simulink model "wscc9_lfc_governor"  (R2024b)
settings: Solver=VariableStepAuto  StartTime=0.0  StopTime=60  MaxStep=0.01  RelTol=1e-3
InitFcn:
  | wscc9_lfc_init
values from neighbouring files (symbols this model uses):
  D = 4    [wscc9_lfc_init.m]
  D10 = del(1)    [wscc9_transient_init.m]
  D20 = del(2)    [wscc9_transient_init.m]
  D30 = del(3)    [wscc9_transient_init.m]
  E1 = E(1)    [wscc9_transient_init.m]
  E2 = E(2)    [wscc9_transient_init.m]
  E3 = E(3)    [wscc9_transient_init.m]
  f = 60    [wscc9_transient_init.m]
  H = [23.645 ; 6.4 ; 3.01]    [wscc9_transient_init.m]
  kS = S_MVA / S_base    [wscc9_lfc_init.m]
  Pm0 = Pe0    [wscc9_lfc_init.m]
  R = 0.05    [wscc9_lfc_init.m]    (also in wscc9_transient_init.m = linedataa(:,3))
  S_base = 100    [wscc9_lfc_init.m]
  t_step = 1    [wscc9_lfc_init.m]
  Tg = 0.2    [wscc9_lfc_init.m]
  Tt = 0.5    [wscc9_lfc_init.m]
  ws = 2*pi*f    [wscc9_lfc_init.m]
  Ypost = kron_reduce(Ystep, 3)    [wscc9_lfc_init.m]
  Ypre = Y1    [wscc9_lfc_init.m]
Description:
  | WSCC 3-machine 9-bus system: load-frequency study (classical SG, model 0.0, with a simple governor)
  | Run: wscc9_lfc_plot (simulates and plots), or press Run. InitFcn = wscc9_lfc_init.m sets every parameter.
  | Units: powers in pu on 100 MVA (MW in the measurement area), dw in rad/s, delta in rad, f in Hz.
  | Swing equation (each SG): d(dw)/dt = (pi f / H)(Pm - Pe - D kS dw/ws),   d(delta)/dt = dw
  | Governor (each SG): dPm = -(kS / R)(dw/ws) -> 1/(1 + s Tg) -> 1/(1 + s Tt),   Pm = Pm0 + dPm   (R = 0.05, Tg = 0.2 s, Tt = 0.5 s, D = 4)
  | Network: Pe_k = sum_j E_k E_j |Y_kj| cos(theta_kj - delta_k + delta_j);  Y switches from Ypre to Ypost at t_step (load step dP_L_MW at step_bus).
  | Goto/From tags: del1-3 = rotor angles, Pe1pre/Pe1post... = Pe before/after the step, w1-3 = dw, Pm1-3, Pe1-3 = measurement taps.
settings Model: Creator=Hussain  LastModifiedBy=Hussain
settings SolverCC: AlgebraicLoopSolver=TrustRegion
settings DebuggingCC: UnconnectedInputMsg=warning  UnconnectedOutputMsg=warning  UnconnectedLineMsg=warning  ArithmeticOperatorsInVariantConditions=warning
settings ModelReferenceCC: EnableRefExpFcnMdlSchedulingChecks=on
settings SFSimCC: SimUseLocalCustomCode=off  CustomCodeUndefinedFunction=UseInterfaceOnly
settings RTWCC: RTWUseLocalCustomCode=off  GPUComputeCapability=3.5
settings CodeAppCC: StateflowObjectComments=on

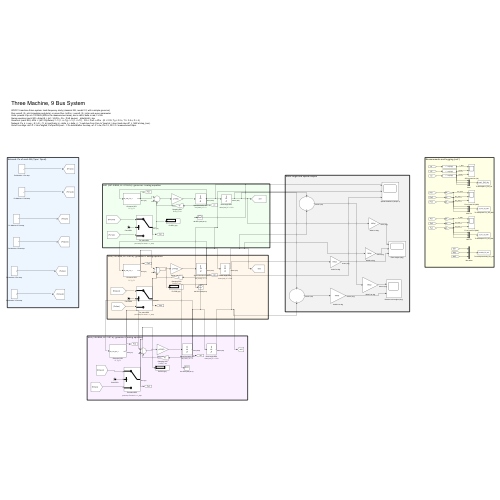
[thumbnail: Simulink's stored preview of the top-level diagram]
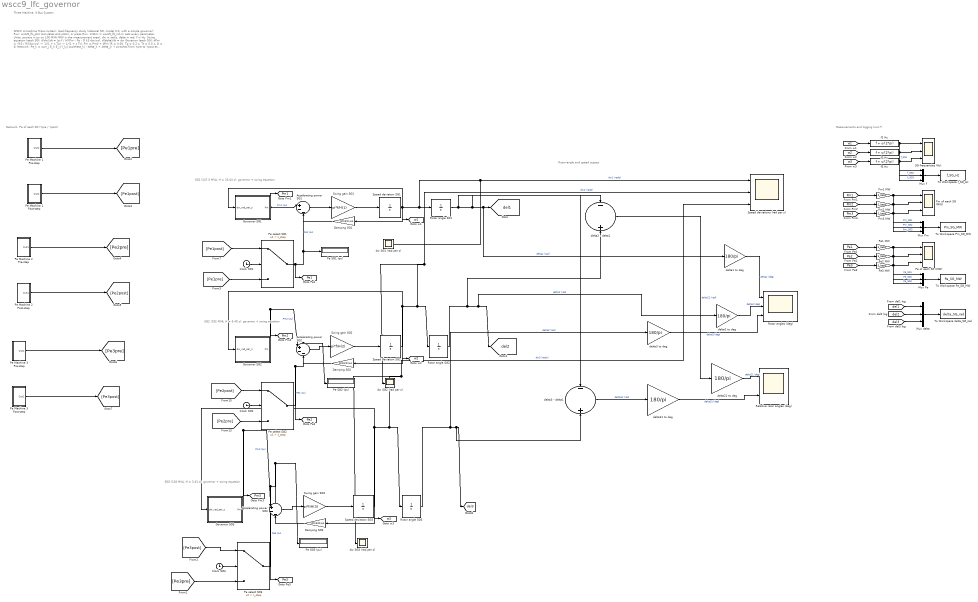
== system wscc9_lfc_governor ==
  note: Three Machine, 9 Bus System
  note: Network: Pe of each SG (Ypre / Ypost)
  note: SG1 (247.5 MVA, H = 23.64 s): governor + swing equation
  note: SG2 (192 MVA, H = 6.40 s): governor + swing equation
  note: SG3 (128 MVA, H = 3.01 s): governor + swing equation
  note: Rotor-angle and speed scopes
  note: Measurements and logging (out.*)
  note: WSCC 3-machine 9-bus system: load-frequency study (classical SG, model 0.0, with a simple governor)
      | Run: wscc9_lfc_plot (simulates and plots), or press Run. InitFcn = wscc9_lfc_init.m sets every parameter.
      | Units: powers in pu on 100 MVA (MW in the measurement area), dw in rad/s, delta in rad, f in Hz.
      | Swing equation (each SG): d(dw)/dt = (pi f / H)(Pm - Pe - D kS dw/ws),   d(delta)/dt = dw
      | Governor (each SG): dPm = -(kS / R)(dw/ws) -> 1/(1 + s Tg) -> 1/(1 + s Tt),   Pm = Pm0 + dPm   (R = 0.05, Tg = 0.2 s, Tt = 0.5 s, D = 4)
      | Network: Pe_k = sum_j E_k E_j |Y_kj| cos(theta_kj - delta_k + delta_j);  Y switches from Ypre to Ypost at t_step (load step dP_L_MW at step_bus).
      | Goto/From tags: del1-3 = rotor angles, Pe1pre/Pe1post... = Pe before/after the step, w1-3 = dw, Pm1-3, Pe1-3 = measurement taps.
  Accelerating power SG1 : Sum  Inputs=|+--
  Accelerating power SG2 : Sum  Inputs=|+--
  Accelerating power SG3 : Sum  Inputs=|+--
  Clock SG1 : Clock
  Clock SG2 : Clock
  Clock SG3 : Clock
  Damping SG1 : Gain  Gain=D*kS(1)/ws
      settings: AttributesFormatString=D kS(1) / ws
  Damping SG2 : Gain  Gain=D*kS(2)/ws
      settings: AttributesFormatString=D kS(2) / ws
  Damping SG3 : Gain  Gain=D*kS(3)/ws
      settings: AttributesFormatString=D kS(3) / ws
  Governor SG1 : Subsystem  Description=Simple non-reheat governor: dPm = -(kS/R)(dw/ws) -> 1/(1+sTg) -> 1/(1+sTt); Pm = Pm0 + dPm [pu, 100 MVA]
      settings: AttributesFormatString=R, Tg, Tt
  Governor SG2 : Subsystem  Description=Simple non-reheat governor: dPm = -(kS/R)(dw/ws) -> 1/(1+sTg) -> 1/(1+sTt); Pm = Pm0 + dPm [pu, 100 MVA]
      settings: AttributesFormatString=R, Tg, Tt
  Governor SG3 : Subsystem  Description=Simple non-reheat governor: dPm = -(kS/R)(dw/ws) -> 1/(1+sTg) -> 1/(1+sTt); Pm = Pm0 + dPm [pu, 100 MVA]
      settings: AttributesFormatString=R, Tg, Tt
  Mux Pe : Mux  Inputs=3
  Mux Pm : Mux  Inputs=3
  Mux delta : Mux  Inputs=3
  Mux f : Mux  Inputs=3
  Pe Machine 1 Post-step : Subsystem  Description=|
      | Electrical power of SG1, post-step network (Ypost):
      | Pe1 = sum over j of  E1 Ej |Ypost(1,j)| cos(theta_1j - delta1 + delta_j),   j = 1..3   [pu, 100 MVA]
      | Constant blocks: E_j and Ypost(1,j); From blocks: rotor angles del1-3; Complex to Magnitude-Angle gives |Y| and theta.
  Pe Machine 1 Pre-step : Subsystem  Description=|
      | Electrical power of SG1, pre-step network (Ypre):
      | Pe1 = sum over j of  E1 Ej |Ypre(1,j)| cos(theta_1j - delta1 + delta_j),   j = 1..3   [pu, 100 MVA]
      | Constant blocks: E_j and Ypre(1,j); From blocks: rotor angles del1-3; Complex to Magnitude-Angle gives |Y| and theta.
  Pe Machine 2 Post-step : Subsystem  Description=|
      | Electrical power of SG2, post-step network (Ypost):
      | Pe2 = sum over j of  E2 Ej |Ypost(2,j)| cos(theta_2j - delta2 + delta_j),   j = 1..3   [pu, 100 MVA]
      | Constant blocks: E_j and Ypost(2,j); From blocks: rotor angles del1-3; Complex to Magnitude-Angle gives |Y| and theta.
  Pe Machine 2 Pre-step : Subsystem  Description=|
      | Electrical power of SG2, pre-step network (Ypre):
      | Pe2 = sum over j of  E2 Ej |Ypre(2,j)| cos(theta_2j - delta2 + delta_j),   j = 1..3   [pu, 100 MVA]
      | Constant blocks: E_j and Ypre(2,j); From blocks: rotor angles del1-3; Complex to Magnitude-Angle gives |Y| and theta.
  Pe Machine 3 Post-step : Subsystem  Description=|
      | Electrical power of SG3, post-step network (Ypost):
      | Pe3 = sum over j of  E3 Ej |Ypost(3,j)| cos(theta_3j - delta3 + delta_j),   j = 1..3   [pu, 100 MVA]
      | Constant blocks: E_j and Ypost(3,j); From blocks: rotor angles del1-3; Complex to Magnitude-Angle gives |Y| and theta.
  Pe Machine 3 Pre-step : Subsystem  Description=|
      | Electrical power of SG3, pre-step network (Ypre):
      | Pe3 = sum over j of  E3 Ej |Ypre(3,j)| cos(theta_3j - delta3 + delta_j),   j = 1..3   [pu, 100 MVA]
      | Constant blocks: E_j and Ypre(3,j); From blocks: rotor angles del1-3; Complex to Magnitude-Angle gives |Y| and theta.
  Pe SG1 (pu) : Display
  Pe SG2 (pu) : Display
  Pe SG3 (pu) : Display
  Pe of each SG (MW) : Scope  NumInputPorts=3
  Pe select SG1 : Switch  Criteria=u2 > Threshold  Threshold=t_step  SaturateOnIntegerOverflow=off  InputSameDT=off
      settings: AttributesFormatString=post-step Pe when t > t_step
  Pe select SG2 : Switch  Criteria=u2 > Threshold  Threshold=t_step  SaturateOnIntegerOverflow=off  InputSameDT=off
      settings: AttributesFormatString=post-step Pe when t > t_step
  Pe select SG3 : Switch  Criteria=u2 > Threshold  Threshold=t_step  SaturateOnIntegerOverflow=off  InputSameDT=off
      settings: AttributesFormatString=post-step Pe when t > t_step
  Pe1 MW : Gain  Gain=S_base
  Pe2 MW : Gain  Gain=S_base
  Pe3 MW : Gain  Gain=S_base
  Pm of each SG (MW) : Scope  NumInputPorts=3
  Pm1 MW : Gain  Gain=S_base
  Pm2 MW : Gain  Gain=S_base
  Pm3 MW : Gain  Gain=S_base
  Relative rotor angles (deg) : Scope  NumInputPorts=2
  Rotor angle SG1 : Integrator  InitialCondition=D10
      settings: AttributesFormatString=delta [rad], IC = %<InitialCondition>
  Rotor angle SG2 : Integrator  InitialCondition=D20
      settings: AttributesFormatString=delta [rad], IC = %<InitialCondition>
  Rotor angle SG3 : Integrator  InitialCondition=D30
      settings: AttributesFormatString=delta [rad], IC = %<InitialCondition>
  Rotor angles (deg) : Scope  NumInputPorts=3
  SG frequencies (Hz) : Scope  NumInputPorts=3
  Speed deviation SG1 : Integrator
      settings: AttributesFormatString=dw [rad/s], IC = 0
  Speed deviation SG2 : Integrator
      settings: AttributesFormatString=dw [rad/s], IC = 0
  Speed deviation SG3 : Integrator
      settings: AttributesFormatString=dw [rad/s], IC = 0
  Speed deviations (rad per s) : Scope  NumInputPorts=3
  Swing gain SG1 : Gain  Gain=pi*f/H(1)
  Swing gain SG2 : Gain  Gain=pi*f/H(2)
  Swing gain SG3 : Gain  Gain=pi*f/H(3)
  To Workspace Pe_SG_MW : ToWorkspace  VariableName=Pe_SG_MW  SaveFormat=Timeseries  SampleTime=-1
  To Workspace Pm_SG_MW : ToWorkspace  VariableName=Pm_SG_MW  SaveFormat=Timeseries  SampleTime=-1
  To Workspace delta_SG_rad : ToWorkspace  VariableName=delta_SG_rad  SaveFormat=Timeseries  SampleTime=-1
  To Workspace f_SG_Hz : ToWorkspace  VariableName=f_SG_Hz  SaveFormat=Timeseries  SampleTime=-1
  delta1 to deg : Gain  Gain=180/pi
  delta2 - delta1 : Sum  Inputs=-+
  delta2 to deg : Gain  Gain=180/pi
  delta21 to deg : Gain  Gain=180/pi
  delta3 - delta1 : Sum  Inputs=-+
  delta3 to deg : Gain  Gain=180/pi
  delta31 to deg : Gain  Gain=180/pi
  dw SG1 (rad per s) : Scope
  dw SG2 (rad per s) : Scope
  dw SG3 (rad per s) : Scope
  f1 Hz : Fcn  Expr=f + u/(2*pi)
  f2 Hz : Fcn  Expr=f + u/(2*pi)
  f3 Hz : Fcn  Expr=f + u/(2*pi)
  tag scope: Pe1=global, Pe2=global, Pe3=global, Pm1=global, Pm2=global, Pm3=global, del1=global, del2=global, del3=global, w1=global, w2=global, w3=global
  wires:
  Speed deviation SG1/1 -> Speed deviations (rad per s)/1, dw SG1 (rad per s)/1, Rotor angle SG1/1, Governor SG1/1(dw_rad_per_s), Damping SG1/1, [w1]  "dw1 (rad/s)"
  Swing gain SG1/1 -> Speed deviation SG1/1
  Accelerating power SG1/1 -> Swing gain SG1/1
  Pe select SG1/1 -> Pe SG1 (pu)/1, Accelerating power SG1/2, [Pe1]  "Pe1 (pu)"
  Clock SG1/1 -> Pe select SG1/2
  Rotor angle SG1/1 -> delta3 - delta1/1, delta2 - delta1/1, delta1 to deg/1, [del1]  "delta1 (rad)"
  Swing gain SG2/1 -> Speed deviation SG2/1
  Accelerating power SG2/1 -> Swing gain SG2/1
  Pe select SG2/1 -> Pe SG2 (pu)/1, Accelerating power SG2/2, [Pe2]  "Pe2 (pu)"
  [Pe2post] -> Pe select SG2/1
  [Pe2pre] -> Pe select SG2/3
  Clock SG2/1 -> Pe select SG2/2
  Rotor angle SG2/1 -> delta2 - delta1/2, delta2 to deg/1, [del2]  "delta2 (rad)"
  [Pe1pre] -> Pe select SG1/3
  [Pe1post] -> Pe select SG1/1
  Pe Machine 1 Pre-step/1(Out1) -> [Pe1pre]
  Pe Machine 1 Post-step/1(Out1) -> [Pe1post]
  Speed deviation SG3/1 -> Speed deviations (rad per s)/3, dw SG3 (rad per s)/1, Rotor angle SG3/1, Governor SG3/1(dw_rad_per_s), Damping SG3/1, [w3]  "dw3 (rad/s)"
  Swing gain SG3/1 -> Speed deviation SG3/1
  Accelerating power SG3/1 -> Swing gain SG3/1
  Pe select SG3/1 -> Accelerating power SG3/2, Pe SG3 (pu)/1, [Pe3]  "Pe3 (pu)"
  Clock SG3/1 -> Pe select SG3/2
  Rotor angle SG3/1 -> delta3 to deg/1, delta3 - delta1/2, [del3]  "delta3 (rad)"
  Pe Machine 2 Pre-step/1(Out1) -> [Pe2pre]
  Pe Machine 2 Post-step/1(Out1) -> [Pe2post]
  Pe Machine 3 Pre-step/1(Out1) -> [Pe3pre]
  Pe Machine 3 Post-step/1(Out1) -> [Pe3post]
  [Pe3pre] -> Pe select SG3/3
  [Pe3post] -> Pe select SG3/1
  delta2 - delta1/1 -> delta21 to deg/1  "delta21 (rad)"
  delta3 - delta1/1 -> delta31 to deg/1  "delta31 (rad)"
  Speed deviation SG2/1 -> Speed deviations (rad per s)/2, dw SG2 (rad per s)/1, Rotor angle SG2/1, Governor SG2/1(dw_rad_per_s), Damping SG2/1, [w2]  "dw2 (rad/s)"
  delta31 to deg/1 -> Relative rotor angles (deg)/2  "delta31 (deg)"
  delta21 to deg/1 -> Relative rotor angles (deg)/1  "delta21 (deg)"
  delta1 to deg/1 -> Rotor angles (deg)/1  "delta1 (deg)"
  delta2 to deg/1 -> Rotor angles (deg)/2  "delta2 (deg)"
  delta3 to deg/1 -> Rotor angles (deg)/3  "delta3 (deg)"
  Governor SG1/1(Pm) -> Accelerating power SG1/1, [Pm1]  "Pm1 (pu)"
  Governor SG2/1(Pm) -> Accelerating power SG2/1, [Pm2]  "Pm2 (pu)"
  Governor SG3/1(Pm) -> Accelerating power SG3/1, [Pm3]  "Pm3 (pu)"
  Damping SG1/1 -> Accelerating power SG1/3
  Damping SG2/1 -> Accelerating power SG2/3
  Damping SG3/1 -> Accelerating power SG3/3
  Mux f/1 -> To Workspace f_SG_Hz/1
  [w1] -> f1 Hz/1
  f1 Hz/1 -> SG frequencies (Hz)/1, Mux f/1  "f_SG1"
  [w2] -> f2 Hz/1
  f2 Hz/1 -> SG frequencies (Hz)/2, Mux f/2  "f_SG2"
  [w3] -> f3 Hz/1
  f3 Hz/1 -> SG frequencies (Hz)/3, Mux f/3  "f_SG3"
  Mux Pm/1 -> To Workspace Pm_SG_MW/1
  [Pm1] -> Pm1 MW/1
  Pm1 MW/1 -> Pm of each SG (MW)/1, Mux Pm/1  "Pm_SG1"
  [Pm2] -> Pm2 MW/1
  Pm2 MW/1 -> Pm of each SG (MW)/2, Mux Pm/2  "Pm_SG2"
  [Pm3] -> Pm3 MW/1
  Pm3 MW/1 -> Pm of each SG (MW)/3, Mux Pm/3  "Pm_SG3"
  Mux Pe/1 -> To Workspace Pe_SG_MW/1
  [Pe1] -> Pe1 MW/1
  Pe1 MW/1 -> Pe of each SG (MW)/1, Mux Pe/1  "Pe_SG1"
  [Pe2] -> Pe2 MW/1
  Pe2 MW/1 -> Pe of each SG (MW)/2, Mux Pe/2  "Pe_SG2"
  [Pe3] -> Pe3 MW/1
  Pe3 MW/1 -> Pe of each SG (MW)/3, Mux Pe/3  "Pe_SG3"
  Mux delta/1 -> To Workspace delta_SG_rad/1
  [del1] -> Mux delta/1
  [del2] -> Mux delta/2
  [del3] -> Mux delta/3

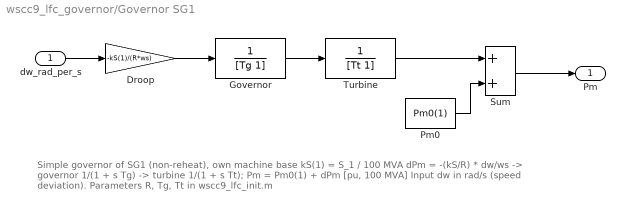
== system wscc9_lfc_governor/Governor SG1 ==
  note: Simple governor of SG1 (non-reheat), own machine base kS(1) = S_1 / 100 MVA
      | dPm = -(kS/R) * dw/ws  ->  governor 1/(1 + s Tg)  ->  turbine 1/(1 + s Tt);   Pm = Pm0(1) + dPm   [pu, 100 MVA]
      | Input dw in rad/s (speed deviation). Parameters R, Tg, Tt in wscc9_lfc_init.m
  dw_rad_per_s : Inport
  Droop : Gain  Gain=-kS(1)/(R*ws)
      settings: AttributesFormatString=-kS(1) / (R ws)
  Governor : TransferFcn  Numerator=1  Denominator=[Tg 1]
      settings: AttributesFormatString=1 / (Tg s + 1)
  Pm0 : Constant  Value=Pm0(1)
  Sum : Sum
  Turbine : TransferFcn  Numerator=1  Denominator=[Tt 1]
      settings: AttributesFormatString=1 / (Tt s + 1)
  Pm : Outport
  wires:
  dw_rad_per_s/1 -> Droop/1
  Droop/1 -> Governor/1
  Governor/1 -> Turbine/1
  Turbine/1 -> Sum/1
  Pm0/1 -> Sum/2
  Sum/1 -> Pm/1

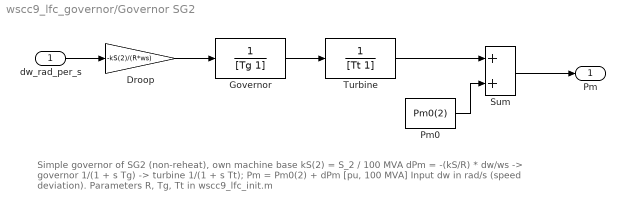
== system wscc9_lfc_governor/Governor SG2 ==
  note: Simple governor of SG2 (non-reheat), own machine base kS(2) = S_2 / 100 MVA
      | dPm = -(kS/R) * dw/ws  ->  governor 1/(1 + s Tg)  ->  turbine 1/(1 + s Tt);   Pm = Pm0(2) + dPm   [pu, 100 MVA]
      | Input dw in rad/s (speed deviation). Parameters R, Tg, Tt in wscc9_lfc_init.m
  dw_rad_per_s : Inport
  Droop : Gain  Gain=-kS(2)/(R*ws)
      settings: AttributesFormatString=-kS(2) / (R ws)
  Governor : TransferFcn  Numerator=1  Denominator=[Tg 1]
      settings: AttributesFormatString=1 / (Tg s + 1)
  Pm0 : Constant  Value=Pm0(2)
  Sum : Sum
  Turbine : TransferFcn  Numerator=1  Denominator=[Tt 1]
      settings: AttributesFormatString=1 / (Tt s + 1)
  Pm : Outport
  wires:
  dw_rad_per_s/1 -> Droop/1
  Droop/1 -> Governor/1
  Governor/1 -> Turbine/1
  Turbine/1 -> Sum/1
  Pm0/1 -> Sum/2
  Sum/1 -> Pm/1

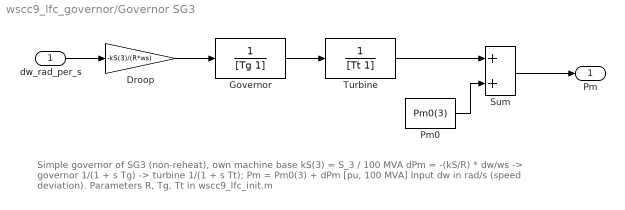
== system wscc9_lfc_governor/Governor SG3 ==
  note: Simple governor of SG3 (non-reheat), own machine base kS(3) = S_3 / 100 MVA
      | dPm = -(kS/R) * dw/ws  ->  governor 1/(1 + s Tg)  ->  turbine 1/(1 + s Tt);   Pm = Pm0(3) + dPm   [pu, 100 MVA]
      | Input dw in rad/s (speed deviation). Parameters R, Tg, Tt in wscc9_lfc_init.m
  dw_rad_per_s : Inport
  Droop : Gain  Gain=-kS(3)/(R*ws)
      settings: AttributesFormatString=-kS(3) / (R ws)
  Governor : TransferFcn  Numerator=1  Denominator=[Tg 1]
      settings: AttributesFormatString=1 / (Tg s + 1)
  Pm0 : Constant  Value=Pm0(3)
  Sum : Sum
  Turbine : TransferFcn  Numerator=1  Denominator=[Tt 1]
      settings: AttributesFormatString=1 / (Tt s + 1)
  Pm : Outport
  wires:
  dw_rad_per_s/1 -> Droop/1
  Droop/1 -> Governor/1
  Governor/1 -> Turbine/1
  Turbine/1 -> Sum/1
  Pm0/1 -> Sum/2
  Sum/1 -> Pm/1

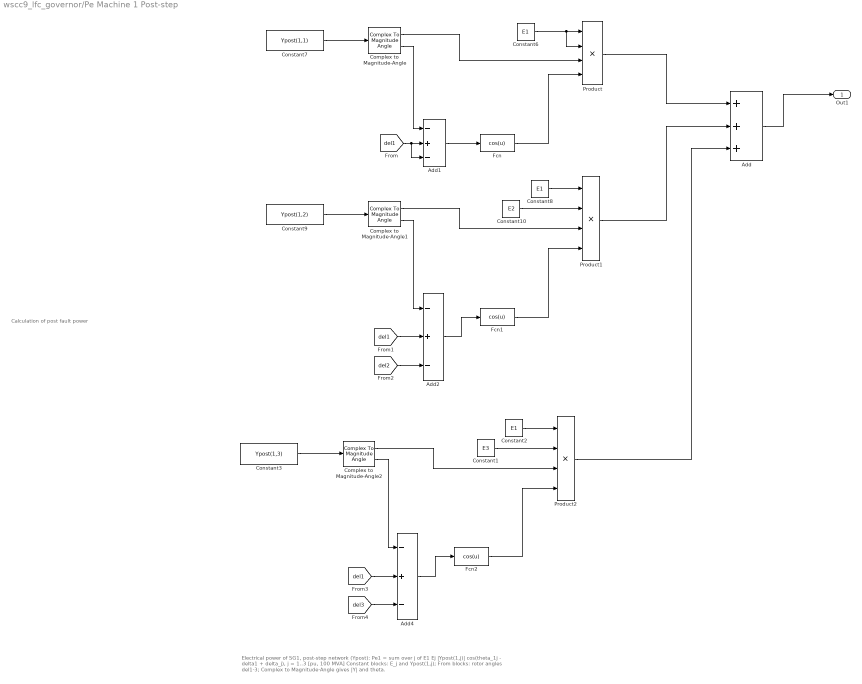
== system wscc9_lfc_governor/Pe Machine 1 Post-step ==
  note: Calculation of post fault power
  note: Electrical power of SG1, post-step network (Ypost):
      | Pe1 = sum over j of  E1 Ej |Ypost(1,j)| cos(theta_1j - delta1 + delta_j),   j = 1..3   [pu, 100 MVA]
      | Constant blocks: E_j and Ypost(1,j); From blocks: rotor angles del1-3; Complex to Magnitude-Angle gives |Y| and theta.
  Add : Sum  Inputs=+++
  Add1 : Sum  Inputs=-+-
  Add2 : Sum  Inputs=-+-
  Add4 : Sum  Inputs=-+-
  Complex to Magnitude-Angle : ComplexToMagnitudeAngle
  Complex to Magnitude-Angle1 : ComplexToMagnitudeAngle
  Complex to Magnitude-Angle2 : ComplexToMagnitudeAngle
  Constant1 : Constant  Value=E3
  Constant10 : Constant  Value=E2
  Constant2 : Constant  Value=E1
  Constant3 : Constant  Value=Ypost(1,3)
  Constant6 : Constant  Value=E1
  Constant7 : Constant  Value=Ypost(1,1)
  Constant8 : Constant  Value=E1
  Constant9 : Constant  Value=Ypost(1,2)
  Fcn : Fcn  Expr=cos(u)
  Fcn1 : Fcn  Expr=cos(u)
  Fcn2 : Fcn  Expr=cos(u)
  Product : Product  Inputs=4
  Product1 : Product  Inputs=4
  Product2 : Product  Inputs=4
  Out1 : Outport
  wires:
  Constant7/1 -> Complex to Magnitude-Angle/1
  Fcn/1 -> Product/4
  Complex to Magnitude-Angle1/1 -> Product1/3
  [del1] -> Add2/2
  Add2/1 -> Fcn1/1
  Complex to Magnitude-Angle1/2 -> Add2/1
  Fcn1/1 -> Product1/4
  Constant8/1 -> Product1/1
  Constant9/1 -> Complex to Magnitude-Angle1/1
  Product1/1 -> Add/2
  Constant6/1 -> Product/2, Product/1
  Add1/1 -> Fcn/1
  Complex to Magnitude-Angle/1 -> Product/3
  Add/1 -> Out1/1
  Product/1 -> Add/1
  [del2] -> Add2/3
  Constant10/1 -> Product1/2
  Complex to Magnitude-Angle/2 -> Add1/1
  [del1] -> Add1/3, Add1/2
  Complex to Magnitude-Angle2/1 -> Product2/3
  [del1] -> Add4/2
  Add4/1 -> Fcn2/1
  Complex to Magnitude-Angle2/2 -> Add4/1
  Fcn2/1 -> Product2/4
  Constant2/1 -> Product2/1
  Constant3/1 -> Complex to Magnitude-Angle2/1
  [del3] -> Add4/3
  Constant1/1 -> Product2/2
  Product2/1 -> Add/3

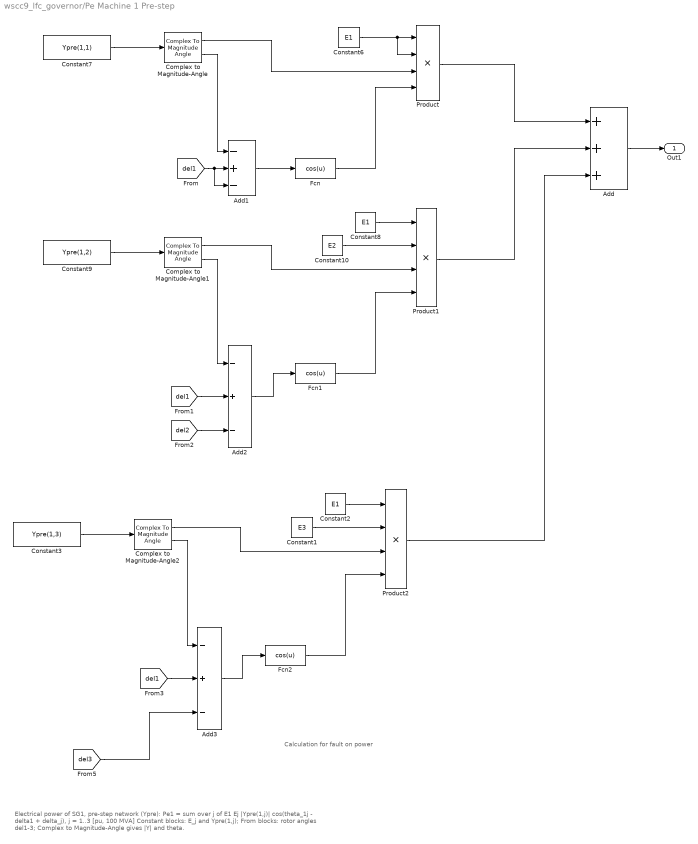
== system wscc9_lfc_governor/Pe Machine 1 Pre-step ==
  note: Calculation for fault on power
  note: Electrical power of SG1, pre-step network (Ypre):
      | Pe1 = sum over j of  E1 Ej |Ypre(1,j)| cos(theta_1j - delta1 + delta_j),   j = 1..3   [pu, 100 MVA]
      | Constant blocks: E_j and Ypre(1,j); From blocks: rotor angles del1-3; Complex to Magnitude-Angle gives |Y| and theta.
  Add : Sum  Inputs=+++
  Add1 : Sum  Inputs=-+-
  Add2 : Sum  Inputs=-+-
  Add3 : Sum  Inputs=-+-
  Complex to Magnitude-Angle : ComplexToMagnitudeAngle
  Complex to Magnitude-Angle1 : ComplexToMagnitudeAngle
  Complex to Magnitude-Angle2 : ComplexToMagnitudeAngle
  Constant1 : Constant  Value=E3
  Constant10 : Constant  Value=E2
  Constant2 : Constant  Value=E1
  Constant3 : Constant  Value=Ypre(1,3)
  Constant6 : Constant  Value=E1
  Constant7 : Constant  Value=Ypre(1,1)
  Constant8 : Constant  Value=E1
  Constant9 : Constant  Value=Ypre(1,2)
  Fcn : Fcn  Expr=cos(u)
  Fcn1 : Fcn  Expr=cos(u)
  Fcn2 : Fcn  Expr=cos(u)
  Product : Product  Inputs=4
  Product1 : Product  Inputs=4
  Product2 : Product  Inputs=4
  Out1 : Outport
  wires:
  Constant7/1 -> Complex to Magnitude-Angle/1
  Fcn/1 -> Product/4
  Complex to Magnitude-Angle1/1 -> Product1/3
  [del1] -> Add2/2
  Add2/1 -> Fcn1/1
  Complex to Magnitude-Angle1/2 -> Add2/1
  Fcn1/1 -> Product1/4
  Constant8/1 -> Product1/1
  Constant9/1 -> Complex to Magnitude-Angle1/1
  Product1/1 -> Add/2
  Constant6/1 -> Product/2, Product/1
  Add1/1 -> Fcn/1
  Complex to Magnitude-Angle/1 -> Product/3
  Add/1 -> Out1/1
  Product/1 -> Add/1
  [del2] -> Add2/3
  Constant10/1 -> Product1/2
  Complex to Magnitude-Angle/2 -> Add1/1
  [del1] -> Add1/3, Add1/2
  Complex to Magnitude-Angle2/1 -> Product2/3
  [del1] -> Add3/2
  Add3/1 -> Fcn2/1
  Complex to Magnitude-Angle2/2 -> Add3/1
  Fcn2/1 -> Product2/4
  Constant2/1 -> Product2/1
  Constant3/1 -> Complex to Magnitude-Angle2/1
  [del3] -> Add3/3
  Constant1/1 -> Product2/2
  Product2/1 -> Add/3

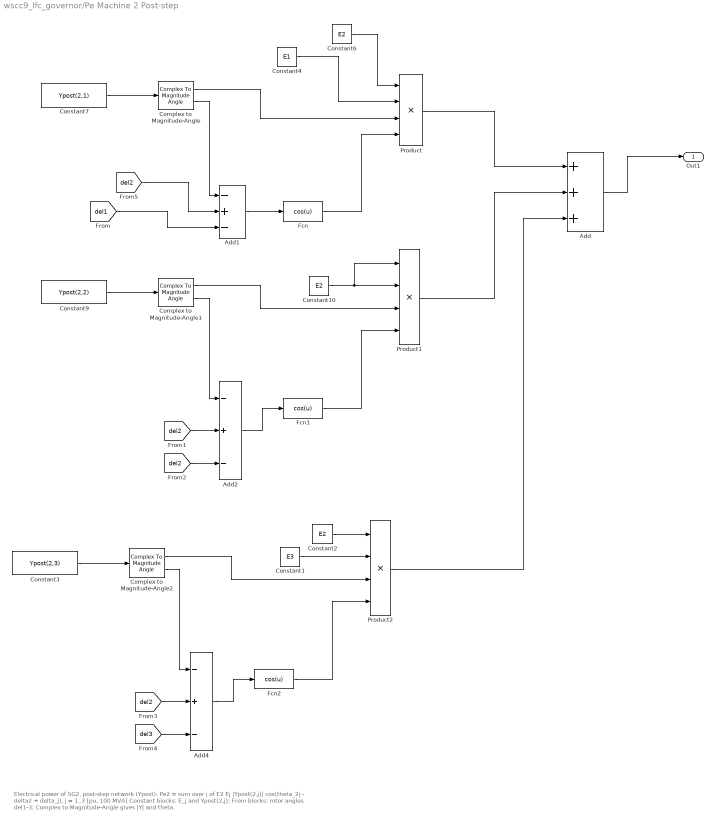
== system wscc9_lfc_governor/Pe Machine 2 Post-step ==
  note: Electrical power of SG2, post-step network (Ypost):
      | Pe2 = sum over j of  E2 Ej |Ypost(2,j)| cos(theta_2j - delta2 + delta_j),   j = 1..3   [pu, 100 MVA]
      | Constant blocks: E_j and Ypost(2,j); From blocks: rotor angles del1-3; Complex to Magnitude-Angle gives |Y| and theta.
  Add : Sum  Inputs=+++
  Add1 : Sum  Inputs=-+-
  Add2 : Sum  Inputs=-+-
  Add4 : Sum  Inputs=-+-
  Complex to Magnitude-Angle : ComplexToMagnitudeAngle
  Complex to Magnitude-Angle1 : ComplexToMagnitudeAngle
  Complex to Magnitude-Angle2 : ComplexToMagnitudeAngle
  Constant1 : Constant  Value=E3
  Constant10 : Constant  Value=E2
  Constant2 : Constant  Value=E2
  Constant3 : Constant  Value=Ypost(2,3)
  Constant4 : Constant  Value=E1
  Constant6 : Constant  Value=E2
  Constant7 : Constant  Value=Ypost(2,1)
  Constant9 : Constant  Value=Ypost(2,2)
  Fcn : Fcn  Expr=cos(u)
  Fcn1 : Fcn  Expr=cos(u)
  Fcn2 : Fcn  Expr=cos(u)
  Product : Product  Inputs=4
  Product1 : Product  Inputs=4
  Product2 : Product  Inputs=4
  Out1 : Outport
  wires:
  Constant7/1 -> Complex to Magnitude-Angle/1
  Fcn/1 -> Product/4
  Complex to Magnitude-Angle1/1 -> Product1/3
  [del2] -> Add2/2
  Add2/1 -> Fcn1/1
  Complex to Magnitude-Angle1/2 -> Add2/1
  Fcn1/1 -> Product1/4
  Constant10/1 -> Product1/1, Product1/2
  Constant9/1 -> Complex to Magnitude-Angle1/1
  Product1/1 -> Add/2
  Constant6/1 -> Product/1
  Add1/1 -> Fcn/1
  Complex to Magnitude-Angle/1 -> Product/3
  Add/1 -> Out1/1
  Product/1 -> Add/1
  [del2] -> Add2/3
  Complex to Magnitude-Angle/2 -> Add1/1
  Complex to Magnitude-Angle2/1 -> Product2/3
  [del2] -> Add4/2
  Add4/1 -> Fcn2/1
  Complex to Magnitude-Angle2/2 -> Add4/1
  Fcn2/1 -> Product2/4
  Constant2/1 -> Product2/1
  Constant3/1 -> Complex to Magnitude-Angle2/1
  [del3] -> Add4/3
  Constant1/1 -> Product2/2
  Product2/1 -> Add/3
  Constant4/1 -> Product/2
  [del1] -> Add1/3
  [del2] -> Add1/2

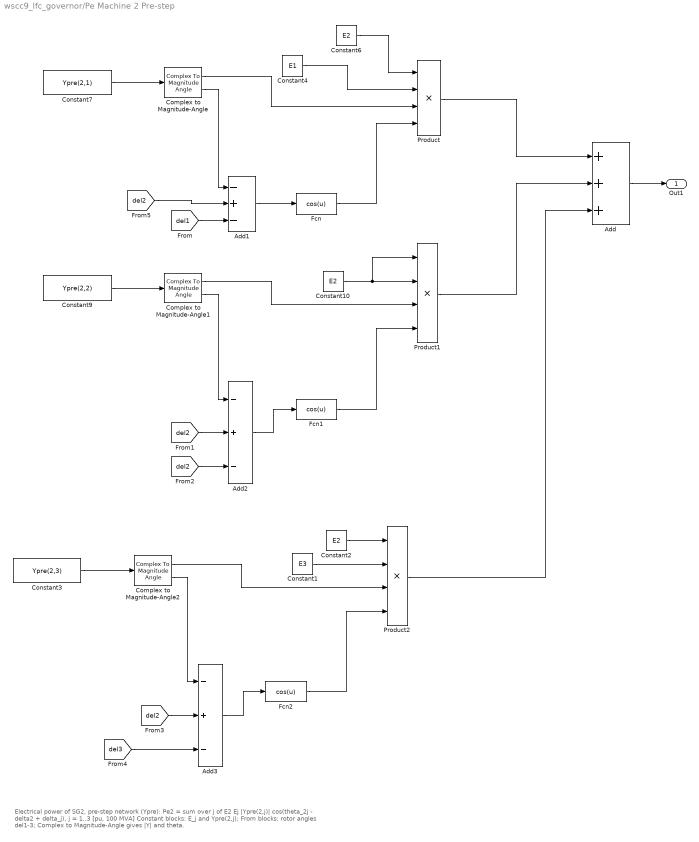
== system wscc9_lfc_governor/Pe Machine 2 Pre-step ==
  note: Electrical power of SG2, pre-step network (Ypre):
      | Pe2 = sum over j of  E2 Ej |Ypre(2,j)| cos(theta_2j - delta2 + delta_j),   j = 1..3   [pu, 100 MVA]
      | Constant blocks: E_j and Ypre(2,j); From blocks: rotor angles del1-3; Complex to Magnitude-Angle gives |Y| and theta.
  Add : Sum  Inputs=+++
  Add1 : Sum  Inputs=-+-
  Add2 : Sum  Inputs=-+-
  Add3 : Sum  Inputs=-+-
  Complex to Magnitude-Angle : ComplexToMagnitudeAngle
  Complex to Magnitude-Angle1 : ComplexToMagnitudeAngle
  Complex to Magnitude-Angle2 : ComplexToMagnitudeAngle
  Constant1 : Constant  Value=E3
  Constant10 : Constant  Value=E2
  Constant2 : Constant  Value=E2
  Constant3 : Constant  Value=Ypre(2,3)
  Constant4 : Constant  Value=E1
  Constant6 : Constant  Value=E2
  Constant7 : Constant  Value=Ypre(2,1)
  Constant9 : Constant  Value=Ypre(2,2)
  Fcn : Fcn  Expr=cos(u)
  Fcn1 : Fcn  Expr=cos(u)
  Fcn2 : Fcn  Expr=cos(u)
  Product : Product  Inputs=4
  Product1 : Product  Inputs=4
  Product2 : Product  Inputs=4
  Out1 : Outport
  wires:
  Constant7/1 -> Complex to Magnitude-Angle/1
  Fcn/1 -> Product/4
  Complex to Magnitude-Angle1/1 -> Product1/3
  [del2] -> Add2/2
  Add2/1 -> Fcn1/1
  Complex to Magnitude-Angle1/2 -> Add2/1
  Fcn1/1 -> Product1/4
  Constant10/1 -> Product1/1, Product1/2
  Constant9/1 -> Complex to Magnitude-Angle1/1
  Product1/1 -> Add/2
  Constant6/1 -> Product/1
  Add1/1 -> Fcn/1
  Complex to Magnitude-Angle/1 -> Product/3
  Add/1 -> Out1/1
  Product/1 -> Add/1
  [del2] -> Add2/3
  Complex to Magnitude-Angle/2 -> Add1/1
  Complex to Magnitude-Angle2/1 -> Product2/3
  [del2] -> Add3/2
  Add3/1 -> Fcn2/1
  Complex to Magnitude-Angle2/2 -> Add3/1
  Fcn2/1 -> Product2/4
  Constant2/1 -> Product2/1
  Constant3/1 -> Complex to Magnitude-Angle2/1
  [del3] -> Add3/3
  Constant1/1 -> Product2/2
  Product2/1 -> Add/3
  Constant4/1 -> Product/2
  [del1] -> Add1/3
  [del2] -> Add1/2

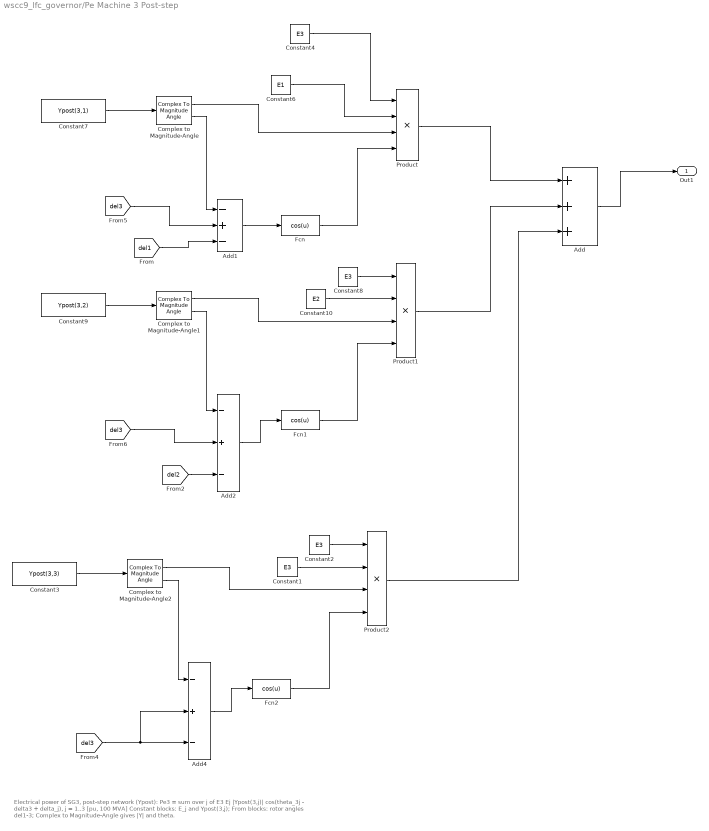
== system wscc9_lfc_governor/Pe Machine 3 Post-step ==
  note: Electrical power of SG3, post-step network (Ypost):
      | Pe3 = sum over j of  E3 Ej |Ypost(3,j)| cos(theta_3j - delta3 + delta_j),   j = 1..3   [pu, 100 MVA]
      | Constant blocks: E_j and Ypost(3,j); From blocks: rotor angles del1-3; Complex to Magnitude-Angle gives |Y| and theta.
  Add : Sum  Inputs=+++
  Add1 : Sum  Inputs=-+-
  Add2 : Sum  Inputs=-+-
  Add4 : Sum  Inputs=-+-
  Complex to Magnitude-Angle : ComplexToMagnitudeAngle
  Complex to Magnitude-Angle1 : ComplexToMagnitudeAngle
  Complex to Magnitude-Angle2 : ComplexToMagnitudeAngle
  Constant{1..2,4,8} (4 alike) : Constant  Value=E3
  Constant10 : Constant  Value=E2
  Constant3 : Constant  Value=Ypost(3,3)
  Constant6 : Constant  Value=E1
  Constant7 : Constant  Value=Ypost(3,1)
  Constant9 : Constant  Value=Ypost(3,2)
  Fcn : Fcn  Expr=cos(u)
  Fcn1 : Fcn  Expr=cos(u)
  Fcn2 : Fcn  Expr=cos(u)
  Product : Product  Inputs=4
  Product1 : Product  Inputs=4
  Product2 : Product  Inputs=4
  Out1 : Outport
  wires:
  Constant7/1 -> Complex to Magnitude-Angle/1
  Fcn/1 -> Product/4
  Complex to Magnitude-Angle1/1 -> Product1/3
  [del3] -> Add2/2
  Add2/1 -> Fcn1/1
  Complex to Magnitude-Angle1/2 -> Add2/1
  Fcn1/1 -> Product1/4
  Constant8/1 -> Product1/1
  Constant9/1 -> Complex to Magnitude-Angle1/1
  Product1/1 -> Add/2
  Add1/1 -> Fcn/1
  Complex to Magnitude-Angle/1 -> Product/3
  Add/1 -> Out1/1
  Product/1 -> Add/1
  [del2] -> Add2/3
  Constant10/1 -> Product1/2
  Complex to Magnitude-Angle/2 -> Add1/1
  [del1] -> Add1/3
  Complex to Magnitude-Angle2/1 -> Product2/3
  [del3] -> Add4/2, Add4/3
  Add4/1 -> Fcn2/1
  Complex to Magnitude-Angle2/2 -> Add4/1
  Fcn2/1 -> Product2/4
  Constant2/1 -> Product2/1
  Constant3/1 -> Complex to Magnitude-Angle2/1
  Constant1/1 -> Product2/2
  Product2/1 -> Add/3
  Constant6/1 -> Product/2
  Constant4/1 -> Product/1
  [del3] -> Add1/2

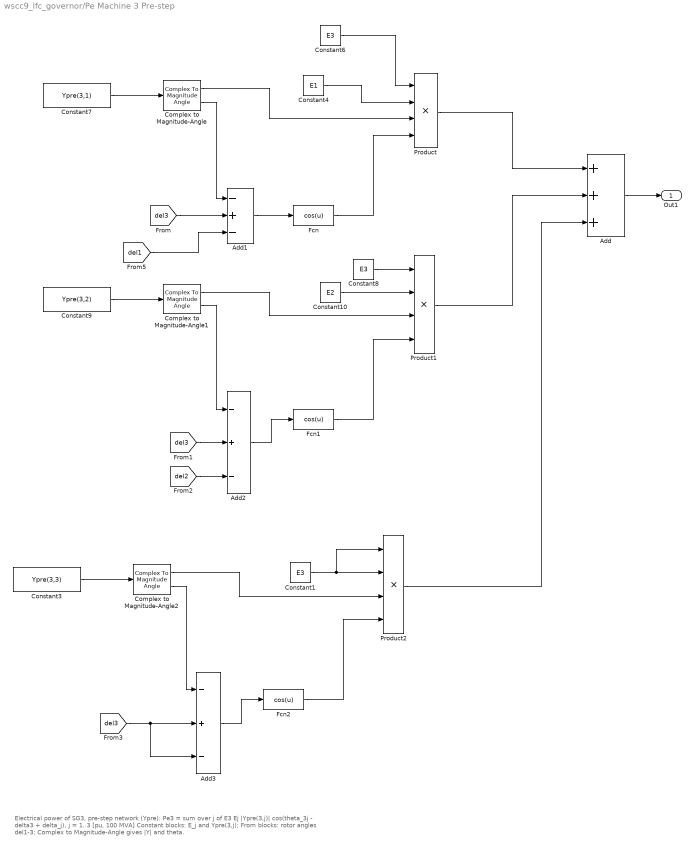
== system wscc9_lfc_governor/Pe Machine 3 Pre-step ==
  note: Electrical power of SG3, pre-step network (Ypre):
      | Pe3 = sum over j of  E3 Ej |Ypre(3,j)| cos(theta_3j - delta3 + delta_j),   j = 1..3   [pu, 100 MVA]
      | Constant blocks: E_j and Ypre(3,j); From blocks: rotor angles del1-3; Complex to Magnitude-Angle gives |Y| and theta.
  Add : Sum  Inputs=+++
  Add1 : Sum  Inputs=-+-
  Add2 : Sum  Inputs=-+-
  Add3 : Sum  Inputs=-+-
  Complex to Magnitude-Angle : ComplexToMagnitudeAngle
  Complex to Magnitude-Angle1 : ComplexToMagnitudeAngle
  Complex to Magnitude-Angle2 : ComplexToMagnitudeAngle
  Constant1 : Constant  Value=E3
  Constant10 : Constant  Value=E2
  Constant3 : Constant  Value=Ypre(3,3)
  Constant4 : Constant  Value=E1
  Constant6 : Constant  Value=E3
  Constant7 : Constant  Value=Ypre(3,1)
  Constant8 : Constant  Value=E3
  Constant9 : Constant  Value=Ypre(3,2)
  Fcn : Fcn  Expr=cos(u)
  Fcn1 : Fcn  Expr=cos(u)
  Fcn2 : Fcn  Expr=cos(u)
  Product : Product  Inputs=4
  Product1 : Product  Inputs=4
  Product2 : Product  Inputs=4
  Out1 : Outport
  wires:
  Constant7/1 -> Complex to Magnitude-Angle/1
  Fcn/1 -> Product/4
  Complex to Magnitude-Angle1/1 -> Product1/3
  [del3] -> Add2/2
  Add2/1 -> Fcn1/1
  Complex to Magnitude-Angle1/2 -> Add2/1
  Fcn1/1 -> Product1/4
  Constant8/1 -> Product1/1
  Constant9/1 -> Complex to Magnitude-Angle1/1
  Product1/1 -> Add/2
  Constant6/1 -> Product/1
  Add1/1 -> Fcn/1
  Complex to Magnitude-Angle/1 -> Product/3
  Add/1 -> Out1/1
  Product/1 -> Add/1
  [del2] -> Add2/3
  Constant10/1 -> Product1/2
  Complex to Magnitude-Angle/2 -> Add1/1
  [del3] -> Add1/2
  Complex to Magnitude-Angle2/1 -> Product2/3
  Add3/1 -> Fcn2/1
  Complex to Magnitude-Angle2/2 -> Add3/1
  Fcn2/1 -> Product2/4
  Constant1/1 -> Product2/1, Product2/2
  Constant3/1 -> Complex to Magnitude-Angle2/1
  [del3] -> Add3/3, Add3/2
  Product2/1 -> Add/3
  Constant4/1 -> Product/2
  [del1] -> Add1/3
